simulink subsystem "Fictious"  (R2024b)
settings: Solver=VariableStepAuto  StartTime=0.0  StopTime=10.0  RelTol=1e-3
libraries: matrix_library x3
settings Model: Creator=pierb  LastModifiedBy=pierb

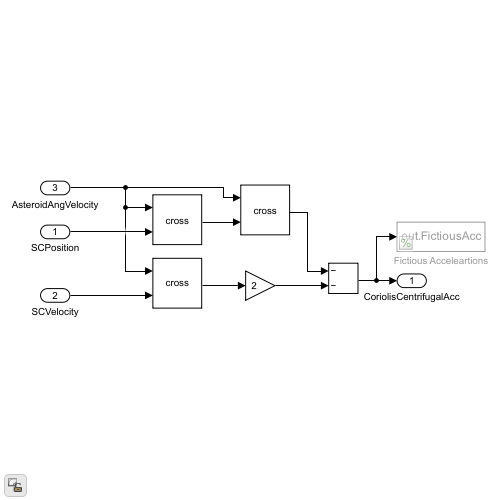
[thumbnail: Simulink's stored preview of the top-level diagram]
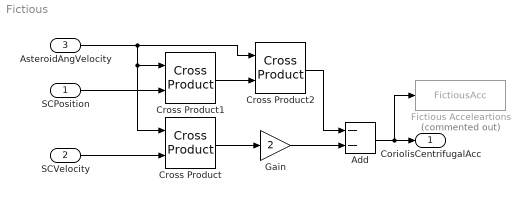
== system Fictious ==
  SCPosition : Inport
  SCVelocity : Inport  Port=2
  AsteroidAngVelocity : Inport  Port=3
  Add : Sum  Inputs=--
  Cross Product : matrix_library/Cross Product
  Cross Product1 : matrix_library/Cross Product
  Cross Product2 : matrix_library/Cross Product
  Fictious Acceleartions : ToWorkspace  Commented=on  VariableName=FictiousAcc  SaveFormat=Timeseries  SampleTime=-1
  Gain : Gain  Gain=2
  CoriolisCentrifugalAcc : Outport
  wires:
  AsteroidAngVelocity/1 -> Cross Product2/1, Cross Product/1, Cross Product1/1
  Cross Product1/1 -> Cross Product2/2
  SCPosition/1 -> Cross Product1/2
  Add/1 -> CoriolisCentrifugalAcc/1, Fictious Acceleartions/1
  SCVelocity/1 -> Cross Product/2
  Cross Product/1 -> Gain/1
  Cross Product2/1 -> Add/1
  Gain/1 -> Add/2
